simulink model "EGR_Adaptive_Fuzzy_Control_FE"  (R2016b)
settings: Solver=FixedStepDiscrete  StartTime=0.0  StopTime=20  FixedStep=0.005  RelTol=1e-3  EnableMultiTasking=on
PreLoadFcn:
  | openecu_make_rtw_hook('model_load', bdroot)
PostLoadFcn:
  | , if any(exist('dsrtsu_mdlpostloadfcn', 'file') == [2, 3, 6]), try dsrtsu_mdlpostloadfcn('Execute', bdroot); catch fprintf('Error in PostLoadFcn (dsrtsu_mdlpostloadfcn) for model "%s":\n %s\n', bdroot, lasterr); end, end,
  | openecu_make_rtw_hook('model_loaded', bdroot)
InitFcn:
  | openecu_make_rtw_hook('model_init', bdroot)
undefined symbols (not defined in the file or in its folder): DiscIntNeverNeededParam
libraries: simulink x6, simulink_extras x1
settings Model: DSRTSU_INTERNAL_RTI_VER=420  DSRTSU_INTERNAL_RTI_TYPE=rti1401  DSRTSU_INTERNAL_RTIFPGA=10  Creator=Andrew Baur  LastModifiedBy=kiebelkx
settings ConfigSet: Description=OpenECU configuration set for code generation under RTW-EC.
settings SolverCC: ZeroCrossControl=DisableAll
settings DataIOCC: LimitDataPoints=on  SaveFormat=Array
settings OptimizationCC: DefaultParameterBehavior=Inlined  InlineInvariantSignals=on  EnhancedBackFolding=on  ExpressionDepthLimit=2147483647  StateBitsets=on  DataBitsets=on  ZeroExternalMemoryAtStartup=off  ZeroInternalMemoryAtStartup=off  NoFixptDivByZeroProtection=on  EfficientFloat2IntCast=on  LifeSpan=1
settings DebuggingCC: AlgebraicLoopMsg=error  SaveWithParameterizedLinksMsg=none  UnderspecifiedInitializationDetection=Classic  MergeDetectMultiDrivingBlocksExec=none  SignalResolutionControl=TryResolveAllWithWarning  MultiTaskDSMMsg=warning  SingleTaskRateTransMsg=error  CheckMatrixSingularityMsg=warning  VectorMatrixConversionMsg=warning  FcnCallInpInsideContextMsg=warning  SignalLabelMismatchMsg=warning  UnconnectedInputMsg=error  UnconnectedLineMsg=error  AllowSymbolicDim=off  StateNameClashWarn=warning  StrictBusMsg=WarnOnBusTreatedAsVector  NonBusSignalsTreatedAsBus=warning  SFUnexpectedBacktrackingDiag=warning  SFNoUnconditionalDefaultTransitionDiag=warning  SFExecutionAtInitializationDiag=none
settings HardwareCC: ProdBitPerPointer=32  ProdBitPerSizeT=32  ProdBitPerPtrDiffT=32  ProdLargestAtomicInteger=Long  ProdLargestAtomicFloat=Double  ProdEndianess=BigEndian  ProdWordSize=32  ProdHWDeviceType=Freescale->32-bit PowerPC  TargetLargestAtomicInteger=Long  TargetLargestAtomicFloat=Double  TargetIntDivRoundTo=Zero  TargetEndianess=BigEndian  TargetHWDeviceType=Freescale->32-bit PowerPC  ProdEqTarget=off
settings ModelReferenceCC: PropagateSignalLabelsOutOfModel=off
settings SFSimCC: SimCustomSourceCode=|
  | /* code to call single float versions of math.h functions instead of double float versions */
  | #define floor(x) floorf(x)
  | #define sqrt(x) sqrtf(x)
  | #define pow(x,y) powf(x,y)
  | #define cos(x) cosf(x)
  | #define sin(x) sinf(x)
  | #define tan(x) tanf(x)
  | #define fabs(x) fabsf(x)
  | #define asin(x) asinf(x)
  | #define acos(x) acosf(x)
  | #define atan(x) atanf(x)
  | #define atan2(x) atan2f(x)
  | #define exp(x) expf(x)
  | #define log10(x) log10f(x)
  | #define log(x) logf(x)
  | #define round(x) roundf(x)
  | #define trunc(x) truncf(x)
  | #define ceil(x) ceilf(x)
  | #define fmod(x,y) fmodf(x,y)
  | #define erf(x) erff(x)
  | #define erfc(x) erfcf(x)
  | #define hypot(x) hypotf(x)
  | #define lgamma(x) lgammaf(x)
  | #define j0(x) j0f(x)
  | #define j1(x) j1f(x)
  | #define jn(x,y) jnf(x,y)
  | #define y0(x) y0f(x)
  | #define y1(x) y1f(x)
  | #define yn(x,y) ynf(x,y)
  | #define ldexp(x,y) ldexpf(x,y)
  | #define frexp(x,y) frexpf(x,y)
  | #define modf(x,y) modff(x,y)
  | #define frexp(x,y) frexpf(x,y)
  | 
  | /* end float code */
settings RTWCC: SystemTargetFile=openecu_ert.tlc  MakeCommand=make_rtw optimized_floating_point=1  TemplateMakefile=openecu_ert_r2016b_64.tmf  Description=OpenECU Platform Target (ERT, optimised floating-point code)  RetainRTWFile=on  IncludeHyperlinkInReport=on
settings RTWCC: CustomSourceCode=|
  | /* code to call single float versions of math.h functions instead of double float versions */
  | #define floor(x) floorf(x)
  | #define sqrt(x) sqrtf(x)
  | #define pow(x,y) powf(x,y)
  | #define cos(x) cosf(x)
  | #define sin(x) sinf(x)
  | #define tan(x) tanf(x)
  | #define fabs(x) fabsf(x)
  | #define asin(x) asinf(x)
  | #define acos(x) acosf(x)
  | #define atan(x) atanf(x)
  | #define atan2(x) atan2f(x)
  | #define exp(x) expf(x)
  | #define log10(x) log10f(x)
  | #define log(x) logf(x)
  | #define round(x) roundf(x)
  | #define trunc(x) truncf(x)
  | #define ceil(x) ceilf(x)
  | #define fmod(x,y) fmodf(x,y)
  | #define erf(x) erff(x)
  | #define erfc(x) erfcf(x)
  | #define hypot(x) hypotf(x)
  | #define lgamma(x) lgammaf(x)
  | #define j0(x) j0f(x)
  | #define j1(x) j1f(x)
  | #define jn(x,y) jnf(x,y)
  | #define y0(x) y0f(x)
  | #define y1(x) y1f(x)
  | #define yn(x,y) ynf(x,y)
  | #define ldexp(x,y) ldexpf(x,y)
  | #define frexp(x,y) frexpf(x,y)
  | #define modf(x,y) modff(x,y)
  | #define frexp(x,y) frexpf(x,y)
  | 
  | /* end float code */
settings CodeAppCC: IgnoreCustomStorageClasses=off  SimulinkDataObjDesc=on  CustomSymbolStrType=$N$R$M  InsertBlockDesc=on  InternalIdentifier=Classic
settings STFCustomTargetCC: TargetLibSuffix=.a  GenerateSampleERTMain=on  IncludeMdlTerminateFcn=off  CombineOutputUpdateFcns=on  IncludeFileDelimiter=UseQuote  ERTCustomFileBanners=on  SupportContinuousTime=off  RemoveResetFunc=on  MATLABClassNameForMDSCustomization=Simulink.SoftwareTarget.ERTCustomization  GRTInterface=off  SystemTargetFile=openecu_ert.tlc
settings ERTTargetCC: GenerateSampleERTMain=on  ParMdlRefBuildCompliant=off  CompOptLevelCompliant=off  ConcurrentExecutionCompliant=off  IncludeMdlTerminateFcn=off  ERTFirstTimeCompliant=off  IncludeFileDelimiter=UseQuote  SupportNonInlinedSFcns=on  ModelStepFunctionPrototypeControlCompliant=off  CPPClassGenCompliant=off  UseToolchainInfoCompliant=off  GenerateASAP2=on  ExtModeMexFile=noextcomm  InlinedParameterPlacement=NonHierarchical  ERTSrcFileBannerTemplate=oe_code_c_template.cgt  ERTHdrFileBannerTemplate=oe_code_h_template.cgt  ERTDataSrcFileTemplate=oe_data_c_template.cgt  ERTDataHdrFileTemplate=oe_data_h_template.cgt  ERTCustomFileTemplate=example_file_process.tlc  GlobalDataDefinition=InSeparateSourceFile  GlobalDataReference=InSeparateHeaderFile  ConvertIfToSwitch=off  SuppressUnreachableDefaultCases=off  EnableUserReplacementTypes=on
settings ConfigComp: CovMetricSettings=dw  CovHtmlReporting=on  CovSaveCumulativeToWorkspaceVar=on  CovSaveSingleToWorkspaceVar=on  CovExternalEMLEnable=off

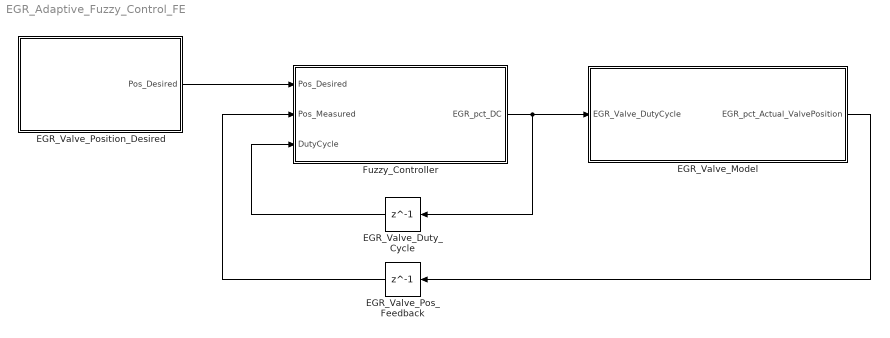
== system EGR_Adaptive_Fuzzy_Control_FE ==
  EGR_Valve_Duty_Cycle : Delay  DelayLength=1  InitialCondition=0
  EGR_Valve_Model : Subsystem
  EGR_Valve_Pos_Feedback : Delay  DelayLength=1  InitialCondition=0
  EGR_Valve_Position_Desired : Subsystem
  Fuzzy_Controller : Subsystem
  wires:
  EGR_Valve_Pos_Feedback/1 -> Fuzzy_Controller/2(Pos_Measured)
  Fuzzy_Controller/1(EGR_pct_DC) -> EGR_Valve_Duty_Cycle/1, EGR_Valve_Model/1(EGR_Valve_DutyCycle)
  EGR_Valve_Model/1(EGR_pct_Actual_ValvePosition) -> EGR_Valve_Pos_Feedback/1
  EGR_Valve_Duty_Cycle/1 -> Fuzzy_Controller/3(DutyCycle)
  EGR_Valve_Position_Desired/1(Pos_Desired) -> Fuzzy_Controller/1(Pos_Desired)

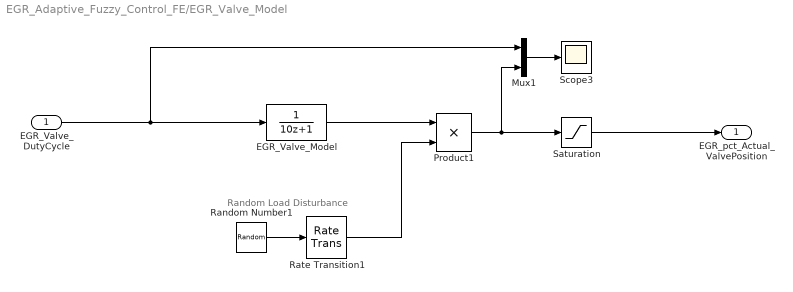
== system EGR_Adaptive_Fuzzy_Control_FE/EGR_Valve_Model ==
  note: Random Load Disturbance
  EGR_Valve_DutyCycle : Inport
  EGR_Valve_Model : DiscreteTransferFcn  Denominator=[10 1]
  Mux1 : Mux  Inputs=2
  Product1 : Product
  Random Number1 : RandomNumber  Mean=12  Variance=8  Seed=10  SampleTime=0.3
  Rate Transition1 : RateTransition
  Saturation : Saturate  UpperLimit=100  LowerLimit=0
  Scope3 : Scope
  EGR_pct_Actual_ValvePosition : Outport
  wires:
  Rate Transition1/1 -> Product1/2
  Random Number1/1 -> Rate Transition1/1
  Mux1/1 -> Scope3/1
  Saturation/1 -> EGR_pct_Actual_ValvePosition/1
  EGR_Valve_Model/1 -> Product1/1
  EGR_Valve_DutyCycle/1 -> EGR_Valve_Model/1, Mux1/1
  Product1/1 -> Mux1/2, Saturation/1

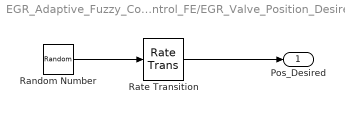
== system EGR_Adaptive_Fuzzy_Control_FE/EGR_Valve_Position_Desired ==
  Random Number : RandomNumber  Mean=50  Variance=100  Seed=50  SampleTime=2
  Rate Transition : RateTransition
  Pos_Desired : Outport
  wires:
  Rate Transition/1 -> Pos_Desired/1
  Random Number/1 -> Rate Transition/1

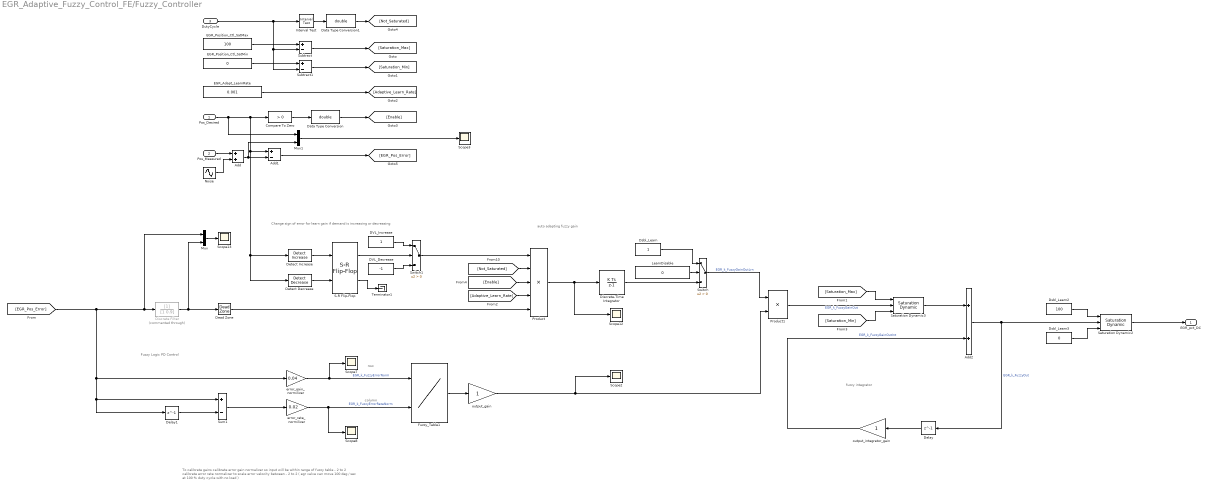
== system EGR_Adaptive_Fuzzy_Control_FE/Fuzzy_Controller ==
  note: Change sign of error for learn gain if demand is increasing or decreasing
  note: Fuzzy Logic PD Control
  note: column
  note: row
  note: auto adapting fuzzy gain
  note: To calibrate gains
      | calibrate error gain normalizer so input will be within range of fuzzy table - 2 to 2
      | calibrate error rate normalizer to scale error velocity between - 2 to 2 ( egr valve can move 100 deg / sec at 100 % duty cycle with no load )
  note: fuzzy integrator
  Pos_Desired : Inport
  Pos_Measured : Inport  Port=2
  DutyCycle : Inport  Port=3
  Add : Sum
  Add1 : Sum  Inputs=+-
  Add2 : Sum
  Compare To Zero : simulink/Logic and Bit Operations/Compare To Zero  relop=>  OutDataTypeStr=boolean
  DVL_Decrease : Constant  Value=-1
  DVL_Increase : Constant
  Data Type Conversion : DataTypeConversion  OutDataTypeStr=double
  Data Type Conversion1 : DataTypeConversion  OutDataTypeStr=double
  Dead Zone : DeadZone  LowerValue=-1  UpperValue=1  SaturateOnIntegerOverflow=on
  Delay : Delay  DelayLength=1  InitialCondition=0
  Delay1 : Delay  DelayLength=1  InitialCondition=0
  Detect Decrease : simulink/Logic and Bit Operations/Detect Decrease  vinit=0.0  OutDataTypeStr=boolean
  Detect Increase : simulink/Logic and Bit Operations/Detect Increase  vinit=0.0  OutDataTypeStr=boolean
  Discrete Filter : DiscreteFilter  Commented=through  Denominator=[1 0.9]
  Discrete-Time Integrator : DiscreteIntegrator  InitialCondition=1  InitialConditionSetting=State (most efficient)  SampleTime=-1  LimitOutput=on  UpperSaturationLimit=2  LowerSaturationLimit=0.5  ICPrevOutput=DiscIntNeverNeededParam  ICPrevScaledInput=DiscIntNeverNeededParam
  Dsbl_Learn : Constant
  Dsbl_Learn2 : Constant  Value=100
  Dsbl_Learn3 : Constant  Value=0
  EGR_Adapt_LearnRate : Constant  Value=0.001  SampleTime=-1
  EGR_Position_Ctl_SatMax : Constant  Value=100  SampleTime=-1
  EGR_Position_Ctl_SatMin : Constant  Value=0  SampleTime=-1
  Fuzzy_Table1 : Lookup_n-D  BreakpointsForDimension1=[-2 -1.8 -1.6 -1.4 -1.2 -1 -0.8 -0.6 -0.4 -0.2 0 0.2 0.4 0.6 0.8 1 1.2 1.4 1.6 1.8 2]  BreakpointsForDimension2=[-2 -1.8 -1.6 -1.4 -1.2 -1 -0.8 -0.6 -0.4 -0.2 0 0.2 0.4 0.6 0.8 1 1.2 1.4 1.6 1.8 2]  Table=[-52 -46.8 -41.6 -36.4 -31.2 -26 -20.8 -15.6 -10.4 -5.2 -5.2 0 0 0 0 0 0 0 0 0 0;-46.8 -42.12 -37.44 -32.76 -28.08 -23.4 -18.72 -14.04 -9.359999999999999 -4.68 -4.68 0 0 0 0 0 0 0 0 0 0;-41.6 -37.44 -33.28 -29.12 -24.96 -20.8 -16.64 -12.48 -8.32 -4.16 -4.16 0 0 0 0 0 0 0 0 0 0;-36.4 -32.76 -29.12 -25.48 -21.84 -18.2 -14.56 -10.92 -7.28 -3.64 -3.64 0 0 0 0 0 0 0 0 0 0;-31.2 -28.08 -24.96 -21.84 -18.72 -15.6 -12.48 -9.359999999999999 -6.24 -3.12 -3.12 0 0 0 0 0 0 0 0 0 0;-26 -23.4 -20.8 -18.2 -15.6 -13 -10.4 -7.8 -5.2 -2.6 -2.6 0 0 0 0 0 0 0 0 0 0;-20.8 -18.72 -16.64 -14.56 -12.48 -10.4 -8.32 -6.24 -4.16 -2.08 -2.08 0 0 0 0 0 0 0 0 0 0;-15.6 -14.04 -12.48 -10.92 -9.359999999999999 -7.8 -6.24 -4.68 -3.12 -1.56 -1.56 0 0 0 0 0 0 0 0 0 0;-10.4 -9.359999999999999 -8.32 -7.28 -6.24 -5.2 -4.16 -3.12 -2.08 -1.04 -1.04 0 0 0 0 0 0 0 0 0 0;-5.2 -4.68 -4.16 -3.64 -3.12 -2.6 -2.08 -1.56 -1.04 -0.52 -0.52 0 0 0 0 0 0 0 0 0 0;0 0 0 0 0 0 0 0 0 0 0 0 0 0 0 0 0 0 0 0 0;0 0 0 0 0 0 0 0 0 0 0.52 0.52 1.04 1.56 2.08 2.6 3.12 3.64 4.16 4.68 5.2;0 0 0 0 0 0 0 0 0 0 1.04 1.04 2.08 3.12 4.16 5.2 6.24 7.28 8.32 9.359999999999999 10.4;0 0 0 0 0 0 0 0 0 0 1.56 1.56 3.12 4.68 6.24 7.8 9.359999999999999 10.92 12.48 14.04 15.6;0 0 0 0 0 0 0 0 0 0 2.08 2.08 4.16 6.24 8.32 10.4 12.48 14.56 16.64 18.72 20.8;0 0 0 0 0 0 0 0 0 0 2.6 2.6 5.2 7.8 10.4 13 15.6 18.2 20.8 23.4 26;0 0 0 0 0 0 0 0 0 0 3.12 3.12 6.24 9.359999999999999 12.48 15.6 18.72 21.84 24.96 28.08 31.2;0 0 0 0 0 0 0 0 0 0 3.64 3.64 7.28 10.92 14.56 18.2 21.84 25.48 29.12 32.76 36.4;0 0 0 0 0 0 0 0 0 0 4.16 4.16 8.32 12.48 16.64 20.8 24.96 29.12 33.28 37.44 41.6;0 0 0 0 0 0 0 0 0 0 4.68 4.68 9.359999999999999 14.04 18.72 23.4 28.08 32.76 37.44 42.12 46.8;0 0 0 0 0 0 0 0 0 0 5.2 5.2 10.4 15.6 20.8 26 31.2 36.4 41.6 46.8 52]  ExtrapMethod=Clip  InternalRulePriority=Speed  RndMeth=Simplest  InputSameDT=on
  Interval Test : simulink/Logic and Bit Operations/Interval Test  IntervalClosedRight=on  uplimit=95  IntervalClosedLeft=on  lowlimit=5  OutDataTypeStr=boolean
  LearnDisable : Constant  Value=0
  Mux : Mux  Inputs=2
  Mux1 : Mux  Inputs=2
  Noise : Sin  Amplitude=0.25  Frequency=5  SampleTime=0.005
  Product : Product  Inputs=5
  Product1 : Product
  S-R Flip-Flop : simulink_extras/Flip Flops/S-R Flip-Flop  initial_condition=0
  Saturation Dynamic2 : simulink/Discontinuities/Saturation Dynamic  OutMin=[]  OutMax=[]  OutDataTypeStr=Inherit: Same as second input  OutDataType=fixdt(1, 16)  OutScaling=2^-10  DoSatur=off
  Saturation Dynamic3 : simulink/Discontinuities/Saturation Dynamic  OutMin=[]  OutMax=[]  OutDataTypeStr=Inherit: Same as second input  OutDataType=fixdt(1, 16)  OutScaling=2^-10  DoSatur=off
  Scope{2..3,7..8,12..13} (6 alike) : Scope
  Subtract : Sum  Inputs=+-
  Subtract1 : Sum  Inputs=+-
  Sum1 : Sum  Inputs=+-
  Switch : Switch  Criteria=u2 > Threshold
  Switch1 : Switch  Criteria=u2 > Threshold
  Terminator1 : Terminator
  error_gain_normilizer : Gain  Gain=0.04
  "error_rate_normilizer " : Gain  Gain=0.02
  output_gain : Gain
  output_integrator_gain : Gain
  EGR_pct_DC : Outport
  wires:
  output_integrator_gain/1 -> Add2/2  "EGR_k_FuzzyGainOutInt"
  Add2/1 -> Delay/1, Saturation Dynamic2/2  "EGR_k_FuzzyOut"
  Delay/1 -> output_integrator_gain/1
  Sum1/1 -> "error_rate_normilizer "/1
  "error_rate_normilizer "/1 -> Scope8/1, Fuzzy_Table1/2  "EGR_k_FuzzyErrorRateNorm"
  Fuzzy_Table1/1 -> output_gain/1
  error_gain_normilizer/1 -> Scope7/1, Fuzzy_Table1/1  "EGR_k_FuzzyErrorNorm"
  output_gain/1 -> Product1/2, Scope2/1
  Delay1/1 -> Sum1/2
  [Adaptive_Learn_Rate] -> Product/4
  Discrete-Time Integrator/1 -> Switch/3
  Compare To Zero/1 -> Data Type Conversion/1
  Product1/1 -> Saturation Dynamic3/2  "EGR_k_FuzzyGainOut"
  Switch/1 -> Product1/1  "EGR_k_FuzzyGainOutLrn"
  Dsbl_Learn/1 -> Switch/1
  LearnDisable/1 -> Switch/2
  EGR_Position_Ctl_SatMax/1 -> Subtract/1
  EGR_Position_Ctl_SatMin/1 -> Subtract1/1
  Subtract/1 -> [Saturation_Max]
  Subtract1/1 -> [Saturation_Min]
  EGR_Adapt_LearnRate/1 -> [Adaptive_Learn_Rate]
  Data Type Conversion/1 -> [Enable]
  [Enable] -> Product/3
  Interval Test/1 -> Data Type Conversion1/1
  Data Type Conversion1/1 -> [Not_Saturated]
  [Not_Saturated] -> Product/2
  [EGR_Pos_Error] -> Mux/1, Discrete Filter/1, error_gain_normilizer/1, Sum1/1, Delay1/1
  Product/1 -> Scope12/1, Discrete-Time Integrator/1
  Discrete Filter/1 -> Dead Zone/1, Mux/2
  Mux/1 -> Scope13/1
  Saturation Dynamic2/1 -> EGR_pct_DC/1
  Dsbl_Learn2/1 -> Saturation Dynamic2/1
  Dsbl_Learn3/1 -> Saturation Dynamic2/3
  [Saturation_Max] -> Saturation Dynamic3/1
  [Saturation_Min] -> Saturation Dynamic3/3
  Saturation Dynamic3/1 -> Add2/1
  Dead Zone/1 -> Product/5
  Pos_Desired/1 -> Mux1/1, Add1/1, Detect Increase/1, Detect Decrease/1, Compare To Zero/1
  Detect Increase/1 -> S-R Flip-Flop/1
  Detect Decrease/1 -> S-R Flip-Flop/2
  S-R Flip-Flop/2 -> Terminator1/1
  S-R Flip-Flop/1 -> Switch1/2
  DVL_Increase/1 -> Switch1/1
  Switch1/1 -> Product/1
  DVL_Decrease/1 -> Switch1/3
  Noise/1 -> Add/2
  Add/1 -> Mux1/2, Add1/2
  DutyCycle/1 -> Subtract1/2, Subtract/2, Interval Test/1
  Pos_Measured/1 -> Add/1
  Add1/1 -> [EGR_Pos_Error]
  Mux1/1 -> Scope3/1
